simulink model "ESWE"  (R2024b)
settings: Solver=FixedStepAuto  StartTime=0.0  StopTime=10.0  RelTol=1e-3
undefined symbols (not defined in the file): DiscIntNeverNeededParam
libraries: dspswit3 x1, spsEdgeDetectorLib x1, eeGeneralControl x1
settings Model: Creator=Student  LastModifiedBy=Student
settings OptimizationCC: DefaultParameterBehavior=Inlined  EnhancedBackFolding=on  PassReuseOutputArgsAs=Individual arguments  ZeroExternalMemoryAtStartup=off  ZeroInternalMemoryAtStartup=off  OptimizeBlockOrder=speed  DifferentSizesBufferReuse=on  OptimizationCustomize=off  EfficientTunableParamExpr=on
settings DebuggingCC: ParameterTunabilityLossMsg=error  SFUnexpectedBacktrackingDiag=warning  SFNoUnconditionalDefaultTransitionDiag=warning
settings HardwareCC: TargetBitPerPointer=64  TargetBitPerSizeT=64  TargetBitPerPtrDiffT=64  TargetLongLongMode=on  TargetIntDivRoundTo=Zero  TargetEndianess=LittleEndian  TargetWordSize=64  TargetHWDeviceType=MATLAB Host  ProdEqTarget=off
settings SFSimCC: MATLABDynamicMemAlloc=off
settings RTWCC: Description=Embedded Coder  SystemTargetFile=ert.tlc  TemplateMakefile=ert_default_tmf  GenerateReport=on  BuildConfiguration=Debug  LaunchReport=on
settings CodeAppCC: ForceParamTrailComments=on  IgnoreCustomStorageClasses=off  OperatorAnnotations=on  SimulinkDataObjDesc=on  SFDataObjDesc=on  InsertBlockDesc=on  EnableCustomComments=on
settings ERTTargetCC: TargetLangStandard=C99 (ISO)  GenerateSampleERTMain=on  SupportContinuousTime=on  ERTCustomFileTemplate=example_file_process.tlc

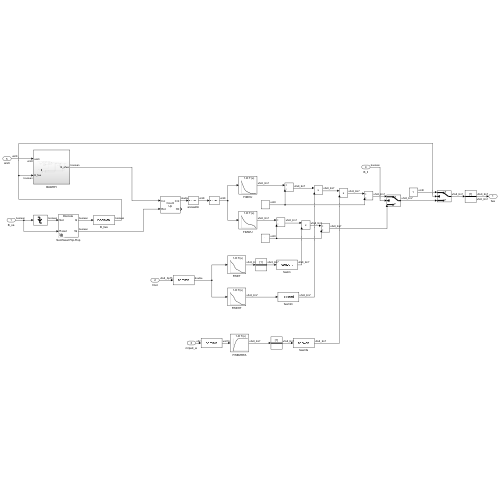
[thumbnail: Simulink's stored preview of the top-level diagram]
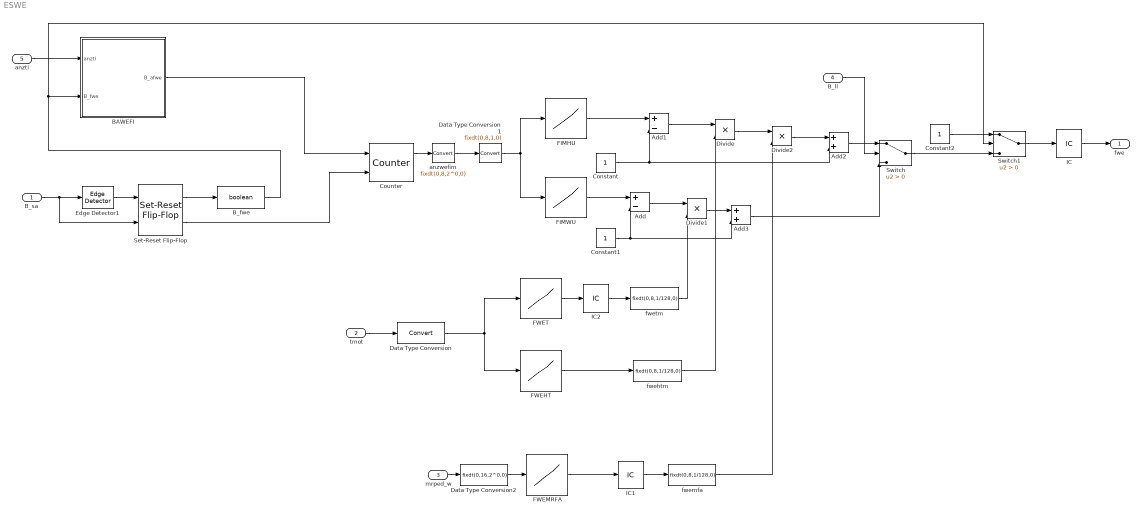
== system ESWE ==
  B_sa : Inport  OutDataTypeStr=boolean
  tmot : Inport  Port=2  OutMin=[-48]  OutMax=[143.5]  OutDataTypeStr=fixdt(0,8,3/4,-48)
  mrped_w : Inport  Port=3  OutMin=[0]  OutMax=[1.99218]  OutDataTypeStr=fixdt(0,16,1/32768,0)
  B_ll : Inport  Port=4  OutDataTypeStr=boolean
  anzti : Inport  Port=5
  Add : Sum  Inputs=+-  OutDataTypeStr=fixdt(0,8,1/128,0)  SaturateOnIntegerOverflow=on
  Add1 : Sum  Inputs=+-  OutDataTypeStr=fixdt(0,8,1/128,0)  SaturateOnIntegerOverflow=on
  Add2 : Sum  OutDataTypeStr=fixdt(0,8,1/128,0)  SaturateOnIntegerOverflow=on
  Add3 : Sum  OutDataTypeStr=fixdt(0,8,1/128,0)  AccumDataTypeStr=fixdt(0,8,1/128,0)  SaturateOnIntegerOverflow=on
  BAWEFI : Subsystem
  B_fwe : DataTypeConversion  OutDataTypeStr=boolean  SaturateOnIntegerOverflow=off  RndMeth=Floor
  Constant : Constant  OutDataTypeStr=uint8
  Constant1 : Constant  OutDataTypeStr=uint8
  Constant2 : Constant  OutDataTypeStr=uint8
  Counter : dspswit3/Counter  Direction=Up  CountEvent=Rising edge  CounterSize=User defined  MaxCount=255  InitialCount=0  Output=Count and Hit  HitValue=32  ResetInput=on  SamplesPerFrame=1  Ts=1  CntDtype=double  HitDtype=Logical
  Data Type Conversion : DataTypeConversion  SaturateOnIntegerOverflow=off  RndMeth=Floor
  Data Type Conversion1 : DataTypeConversion  OutMin=[0]  OutMax=[15]  OutDataTypeStr=fixdt(0,8,1,0)  SaturateOnIntegerOverflow=off  RndMeth=Floor
  Data Type Conversion2 : DataTypeConversion  OutDataTypeStr=fixdt(0,16,2^0,0)  RndMeth=Floor
  Divide : Product  Inputs=**  OutDataTypeStr=fixdt(0,8,1/128,0)  SaturateOnIntegerOverflow=on
  Divide1 : Product  Inputs=**  OutDataTypeStr=fixdt(0,8,1/128,0)  SaturateOnIntegerOverflow=on
  Divide2 : Product  Inputs=**  OutDataTypeStr=fixdt(0,8,1/128,0)  SaturateOnIntegerOverflow=on
  Edge Detector1 : spsEdgeDetectorLib/Edge Detector  model=Falling  ic=0  Ts=0
      settings: LibrarySourceBlock=sps_lib/Control/Edge Detector
  FIMHU : Lookup_n-D  NumberOfTableDimensions=1  BreakpointsForDimension1=[0;1;2;3;4;5;6;7;8;9;10;11;12;13;14;15]  BreakpointsForDimension1DataTypeStr=Inherit: Inherit from 'Breakpoint data'  Table=[1.367187;1.265625;1.195312;1.125;1.085937;1.0625;1.039062;1.023437;1.015625;1;1;1;1;1;1;1]  ExtrapMethod=Clip  InternalRulePriority=Speed  OutMin=[1]  OutMax=[1.99219]  OutDataTypeStr=fixdt(0,8,1/128,0)  RndMeth=Simplest
  FIMWU : Lookup_n-D  NumberOfTableDimensions=1  BreakpointsForDimension1=[0;1;2;3;4;5;6;7;8;9;10;11;12;13;14;15]  BreakpointsForDimension1DataTypeStr=Inherit: Inherit from 'Breakpoint data'  Table=[1.351562;1.289062;1.234375;1.195312;1.164062;1.140625;1.125;1.109375;1.101562;1.101562;1.09375;1.085937;1.078125;1.0625;1.039062;1]  ExtrapMethod=Clip  InternalRulePriority=Speed  OutMin=[1]  OutMax=[1.99219]  OutDataTypeStr=fixdt(0,8,1/128,0)  RndMeth=Simplest
  FWEHT : Lookup_n-D  NumberOfTableDimensions=1  BreakpointsForDimension1=[-30;-20.25;-9.75;0;9.75;20.25;39.75;69.75;90]  Table=[1.476562;1.398437;1.351562;1.289062;1.195312;1.125;1.101562;1;1]  ExtrapMethod=Clip  InternalRulePriority=Speed  OutMin=[0]  OutMax=[1.99219]  OutDataTypeStr=fixdt(0,8,1/128,0)  RndMeth=Simplest
  FWEMRFA : Lookup_n-D  NumberOfTableDimensions=1  BreakpointsForDimension1=[1.9989013671875;4.0008544921875;5.999755859375;7.9986572265625;10.0006103515625;20.001220703125]  Table=[0.601562;0.8125;0.921875;0.984375;1;1]  ExtrapMethod=Clip  InternalRulePriority=Speed  OutMin=[0]  OutMax=[1.99219]  OutDataTypeStr=fixdt(0,8,1/128,0)  RndMeth=Simplest
  FWET : Lookup_n-D  NumberOfTableDimensions=1  BreakpointsForDimension1=[-30;-20.25;-9.75;0;9.75;20.25;39.75;69.75;90]  BreakpointsForDimension1Min=[-48]  BreakpointsForDimension1Max=[143.5]  BreakpointsForDimension1DataTypeStr=Inherit: Inherit from 'Breakpoint data'  Table=[1.476562;1.398437;1.351562;1.289062;1.195312;1.125;1.101562;1;1]  ExtrapMethod=Clip  InternalRulePriority=Speed  OutMin=[0]  OutMax=[1.99219]  OutDataTypeStr=fixdt(0,8,1/128,0)  RndMeth=Simplest
  IC : InitialCondition
  IC1 : InitialCondition
  IC2 : InitialCondition
  Set-Reset Flip-Flop : eeGeneralControl/Set-Reset Flip-Flop  LabelModeActiveChoice=Discrete  UndefState=Set  Q0=0  Ts=-1
      settings: LibrarySourceBlock=ee_sl_lib/General Control/Set-Reset Flip-Flop
  Switch : Switch  Criteria=u2 > Threshold  OutMin=[0]  OutMax=[1.99219]  OutDataTypeStr=fixdt(0,8,1/128,0)  InputSameDT=off
  Switch1 : Switch  Criteria=u2 > Threshold  OutMin=[0]  OutMax=[1.99219]  OutDataTypeStr=fixdt(0,8,1/128,0)  InputSameDT=off
  anzwefim : DataTypeConversion  OutMin=[0]  OutMax=[255]  OutDataTypeStr=fixdt(0,8,2^0,0)  RndMeth=Floor
  fwehtm : DataTypeConversion  OutMin=[0]  OutMax=[1.99219]  OutDataTypeStr=fixdt(0,8,1/128,0)  RndMeth=Floor
  fwemfa : DataTypeConversion  OutMin=[0]  OutMax=[1.99219]  OutDataTypeStr=fixdt(0,8,1/128,0)  RndMeth=Floor
  fwetm : DataTypeConversion  OutMin=[0]  OutMax=[1.99219]  OutDataTypeStr=fixdt(0,8,1/128,0)  RndMeth=Floor
  fwe : Outport  OutMin=[0]  OutMax=[1.99219]  OutDataTypeStr=fixdt(0,8,1/128,0)
  wires:
  B_sa/1 -> Set-Reset Flip-Flop/2, Edge Detector1/1
  Edge Detector1/1 -> Set-Reset Flip-Flop/1
  Set-Reset Flip-Flop/1 -> B_fwe/1
  Set-Reset Flip-Flop/2 -> Counter/2
  B_fwe/1 -> BAWEFI/2(B_fwe), Switch1/2
  Counter/1 -> anzwefim/1
  anzwefim/1 -> Data Type Conversion1/1
  FIMHU/1 -> Add1/1
  Add1/1 -> Divide/1
  Divide/1 -> Divide2/1
  Divide2/1 -> Add2/1
  FIMWU/1 -> Add/1
  Add/1 -> Divide1/1
  Add3/1 -> Switch/3
  Divide1/1 -> Add3/1
  Constant/1 -> Add1/2, Add2/2
  Constant1/1 -> Add3/2, Add/2
  FWET/1 -> IC2/1
  FWEHT/1 -> fwehtm/1
  fwetm/1 -> Divide1/2
  fwehtm/1 -> Divide/2
  FWEMRFA/1 -> IC1/1
  fwemfa/1 -> Divide2/2
  Add2/1 -> Switch/1
  B_ll/1 -> Switch/2
  Constant2/1 -> Switch1/1
  Switch/1 -> Switch1/3
  Switch1/1 -> IC/1
  anzti/1 -> BAWEFI/1(anzti)
  IC2/1 -> fwetm/1
  IC1/1 -> fwemfa/1
  IC/1 -> fwe/1
  BAWEFI/1(B_afwe) -> Counter/1
  mrped_w/1 -> Data Type Conversion2/1
  Data Type Conversion2/1 -> FWEMRFA/1
  tmot/1 -> Data Type Conversion/1
  Data Type Conversion1/1 -> FIMWU/1, FIMHU/1
  Data Type Conversion/1 -> FWEHT/1, FWET/1

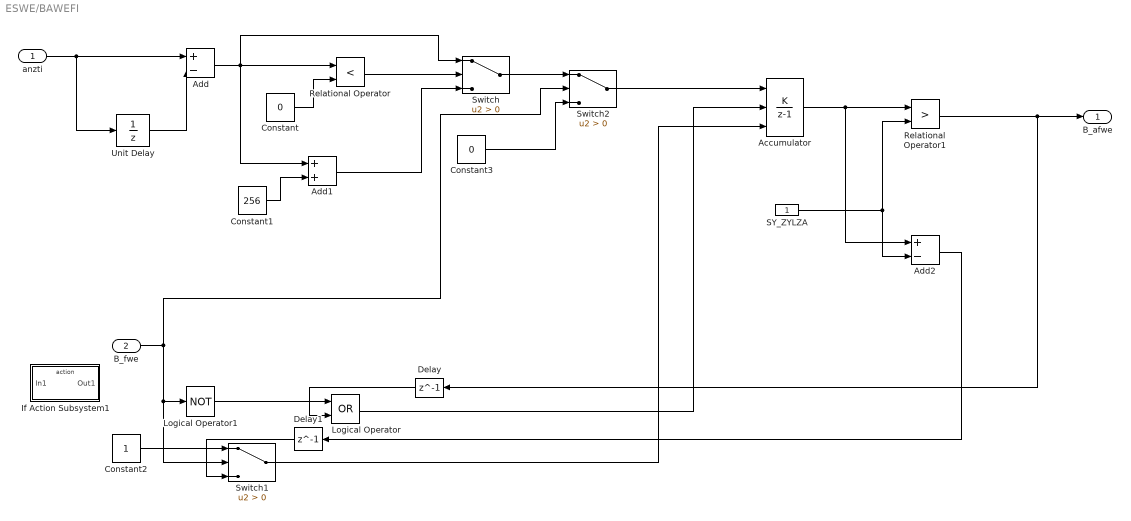
== system ESWE/BAWEFI ==
  anzti : Inport  OutMin=[0]  OutMax=[255]  OutDataTypeStr=uint8
  B_fwe : Inport  Port=2  OutDataTypeStr=boolean
  Accumulator : DiscreteIntegrator  IntegratorMethod=Accumulation: Forward Euler  ExternalReset=rising  InitialConditionSource=external  SampleTime=-1  ICPrevOutput=DiscIntNeverNeededParam  ICPrevScaledInput=DiscIntNeverNeededParam
  Add : Sum  Inputs=+-
  Add1 : Sum
  Add2 : Sum  Inputs=+-
  Constant : Constant  Value=0
  Constant1 : Constant  Value=256
  Constant2 : Constant
  Constant3 : Constant  Value=0
  Delay : Delay  DelayLength=1  InitialCondition=0
  Delay1 : Delay  DelayLength=1  InitialCondition=0
  If Action Subsystem1 : Subsystem  TreatAsAtomicUnit=on
  Logical Operator : Logic  Operator=OR  AllPortsSameDT=off  OutDataTypeStr=boolean
  Logical Operator1 : Logic  Operator=NOT  AllPortsSameDT=off  OutDataTypeStr=boolean
  Relational Operator : RelationalOperator  Operator=<  OutDataTypeStr=boolean  RndMeth=Simplest  InputSameDT=off
  Relational Operator1 : RelationalOperator  Operator=>  OutDataTypeStr=boolean  RndMeth=Simplest  InputSameDT=off
  SY_ZYLZA : Constant
  Switch : Switch  Criteria=u2 > Threshold  SaturateOnIntegerOverflow=off  InputSameDT=off
  Switch1 : Switch  Criteria=u2 > Threshold  SaturateOnIntegerOverflow=off  InputSameDT=off
  Switch2 : Switch  Criteria=u2 > Threshold  SaturateOnIntegerOverflow=off  InputSameDT=off
  Unit Delay : UnitDelay  SampleTime=-1  HasFrameUpgradeWarning=on
  B_afwe : Outport  OutDataTypeStr=boolean
  wires:
  anzti/1 -> Add/1, Unit Delay/1
  Unit Delay/1 -> Add/2
  Add/1 -> Switch/1, Add1/1, Relational Operator/1
  Constant/1 -> Relational Operator/2
  Constant1/1 -> Add1/2
  Relational Operator/1 -> Switch/2
  Add1/1 -> Switch/3
  SY_ZYLZA/1 -> Add2/2, Relational Operator1/2
  Accumulator/1 -> Relational Operator1/1, Add2/1
  Relational Operator1/1 -> B_afwe/1, Delay/1
  Constant2/1 -> Switch1/1
  Add2/1 -> Delay1/1
  Logical Operator1/1 -> Logical Operator/1
  Logical Operator/1 -> Accumulator/2
  Switch1/1 -> Accumulator/3
  Switch/1 -> Switch2/1
  B_fwe/1 -> Switch2/2, Switch1/2, Logical Operator1/1
  Constant3/1 -> Switch2/3
  Switch2/1 -> Accumulator/1
  Delay1/1 -> Switch1/3
  Delay/1 -> Logical Operator/2

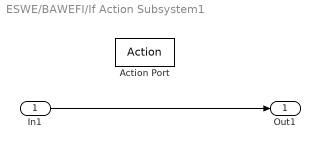
== system ESWE/BAWEFI/If Action Subsystem1 ==
  In1 : Inport
  Action Port : ActionPort
  Out1 : Outport
  wires:
  In1/1 -> Out1/1
